simulink model "temp_control"  (R2022a)
settings: Solver=ode4  StartTime=0.0  StopTime=200  FixedStep=0.1  RelTol=1e-3  EnableMultiTasking=on
libraries: arduinolib x2
settings Model: ExtModeTrigDuration=2  Creator=ryan  LastModifiedBy=ryan
settings OptimizationCC: EnhancedBackFolding=on  PassReuseOutputArgsAs=Individual arguments  ZeroExternalMemoryAtStartup=off  ZeroInternalMemoryAtStartup=off  MaxStackSize=64  OptimizeBlockOrder=speed  DifferentSizesBufferReuse=on  OptimizationCustomize=off  EfficientTunableParamExpr=on
settings DebuggingCC: ParameterTunabilityLossMsg=error
settings HardwareCC: ProdBitPerInt=16  ProdBitPerPointer=16  ProdBitPerSizeT=16  ProdBitPerPtrDiffT=16  ProdLargestAtomicFloat=None  ProdWordSize=8  ProdHWDeviceType=Atmel->AVR
settings SFSimCC: MATLABDynamicMemAlloc=off
settings RTWCC: SystemTargetFile=ert.tlc  HardwareBoard=Arduino Mega 2560  TemplateMakefile=ert_default_tmf  Toolchain=Arduino AVR  BuildConfiguration=Faster Runs
settings CodeAppCC: ForceParamTrailComments=on  IgnoreCustomStorageClasses=off  OperatorAnnotations=on  SimulinkDataObjDesc=on  SFDataObjDesc=on  InsertBlockDesc=on
settings ERTTargetCC: SupportContinuousTime=on  SupportVariableSizeSignals=on  ExtModeTransport=3  ExtModeStaticAlloc=on  ExtModeStaticAllocSize=2048  ExtModeMexFile=ext_xcp  ExtModeIntrfLevel=Level2 - Open

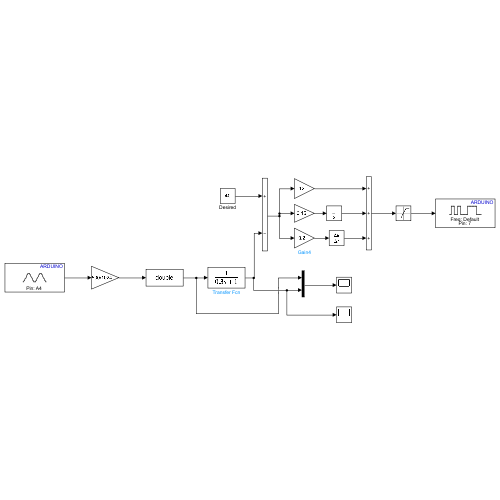
[thumbnail: Simulink's stored preview of the top-level diagram]
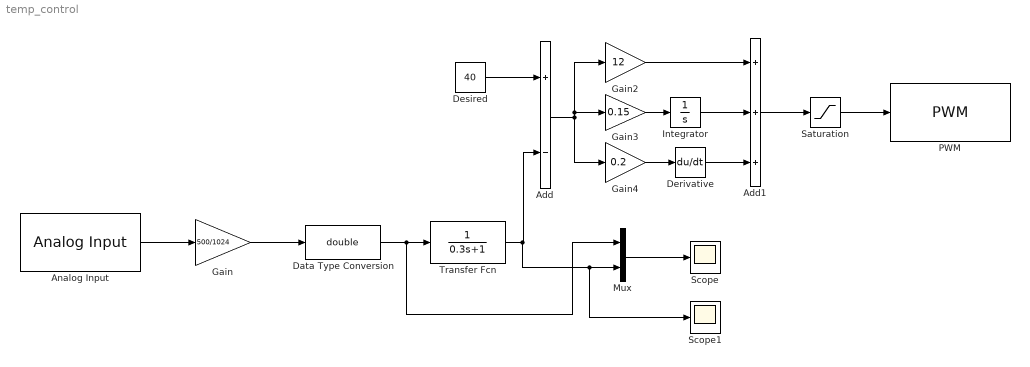
== system temp_control ==
  Add : Sum  Inputs=+-
  Add1 : Sum  Inputs=+++
  Analog Input : arduinolib/Analog Input  pinNumber=4  ReadResultsOnly=off  ConversionTriggerSource=Software  ExternalTriggerType=uint32( 0 )  OutputDataType=uint16  EnableConversionCompleteNotify=off  EnableOuputStatus=off  SampleTime=-1  blockPlatform=arduino
  Data Type Conversion : DataTypeConversion  OutDataTypeStr=double  SaturateOnIntegerOverflow=off  RndMeth=Floor
  Derivative : Derivative
  Desired : Constant  Value=40
  Gain : Gain  Gain=500/1024
  Gain2 : Gain  Gain=12
  Gain3 : Gain  Gain=0.15
  Gain4 : Gain  Gain=0.2
  Integrator : Integrator
  Mux : Mux  Inputs=2
  PWM : arduinolib/PWM  pinNumber=7  frequencyType=Default  desiredFrequency=490.2  achievableFrequency=490.2
  Saturation : Saturate  UpperLimit=255  LowerLimit=0
  Scope : Scope
  Scope1 : Scope
  Transfer Fcn : TransferFcn  Denominator=[0.3 1]
  wires:
  Analog Input/1 -> Gain/1
  Gain/1 -> Data Type Conversion/1
  Data Type Conversion/1 -> Mux/1, Transfer Fcn/1
  Transfer Fcn/1 -> Scope1/1, Mux/2, Add/2
  Desired/1 -> Add/1
  Add/1 -> Gain2/1, Gain3/1, Gain4/1
  Gain3/1 -> Integrator/1
  Gain4/1 -> Derivative/1
  Gain2/1 -> Add1/1
  Integrator/1 -> Add1/2
  Derivative/1 -> Add1/3
  Add1/1 -> Saturation/1
  Saturation/1 -> PWM/1
  Mux/1 -> Scope/1
